simulink model "Driver"  (R2026b)
settings: Solver=VariableStepAuto
undefined symbols (not defined in the file): Driver, Maneuver, Scene, Vehicle, Visual, X, xy_data_car_side, Y, Z
libraries: sm_lib x18, simulink x13, nesl_utility x5, drivingvehiclecontroller x1, autolibshared x1, $bdroot x1
(part 2 of 2)

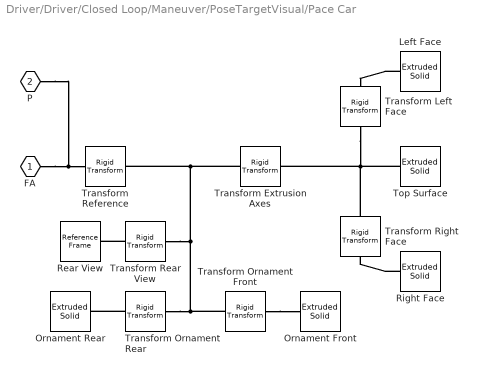
== system Driver/Driver/Closed Loop/Maneuver/PoseTargetVisual/Pace Car ==
  Left Face : sm_lib/Body Elements/Extruded Solid  ExtrusionType=General  PolygonNumSides=3  PolygonOuterRadius=1  PolygonOuterRadiusUnits=m  ExportEntireGeometry=off  ExtrusionCrossSection=xy_data_car_side  ExtrusionCrossSectionUnits=m  ExportConvexHullGeometry=off  ExtrusionLength=thk_side  ExtrusionLengthUnits=m  InertiaType=PointMass  BasedOnType=Density  Density=1000  DensityUnits=kg/m^3  Mass=0  MassUnits=kg  CenterOfMass=[0 0 0]  CenterOfMassUnits=m  MomentsOfInertia=[1 1 1]  MomentsOfInertiaUnits=kg*m^2  ProductsOfInertia=[0 0 0]  ProductsOfInertiaUnits=kg*m^2  GraphicType=FromGeometry  MarkerShape=Sphere  MarkerSize=10  GraphicVisPropType=SimpleVisualProperties  GraphicDiffuseColor=clr_body_geo_left  GraphicOpacity=opc_body_geo_left  GraphicSpecularColor=[0.5 0.5 0.5 1.0]  GraphicAmbientColor=[0.15 0.15 0.15 1.0]  GraphicEmissiveColor=[0.0 0.0 0.0 1.0]  GraphicShininess=75  DoExposeReferenceFrame=on  SerializedFrames=<Frames/>
  Ornament Front : sm_lib/Body Elements/Extruded Solid  ExtrusionType=General  PolygonNumSides=3  PolygonOuterRadius=1  PolygonOuterRadiusUnits=m  ExportEntireGeometry=off  ExtrusionCrossSection=extr_data_emblem_f  ExtrusionCrossSectionUnits=m  ExportConvexHullGeometry=off  ExtrusionLength=0.01  ExtrusionLengthUnits=m  InertiaType=CalculateFromGeometry  BasedOnType=Density  Density=1000  DensityUnits=kg/m^3  Mass=1  MassUnits=kg  CenterOfMass=[0 0 0]  CenterOfMassUnits=m  MomentsOfInertia=[1 1 1]  MomentsOfInertiaUnits=kg*m^2  ProductsOfInertia=[0 0 0]  ProductsOfInertiaUnits=kg*m^2  GraphicType=FromGeometry  MarkerShape=Sphere  MarkerSize=10  GraphicVisPropType=SimpleVisualProperties  GraphicDiffuseColor=clr_emblem_f  GraphicOpacity=opc_emblem_f  GraphicSpecularColor=[0.5 0.5 0.5 1.0]  GraphicAmbientColor=[0.15 0.15 0.15 1.0]  GraphicEmissiveColor=[0.0 0.0 0.0 1.0]  GraphicShininess=75  DoExposeReferenceFrame=on  SerializedFrames=<Frames/>
  Ornament Rear : sm_lib/Body Elements/Extruded Solid  ExtrusionType=General  PolygonNumSides=3  PolygonOuterRadius=1  PolygonOuterRadiusUnits=m  ExportEntireGeometry=off  ExtrusionCrossSection=extr_data_emblem_r  ExtrusionCrossSectionUnits=m  ExportConvexHullGeometry=off  ExtrusionLength=0.01  ExtrusionLengthUnits=m  InertiaType=CalculateFromGeometry  BasedOnType=Density  Density=1000  DensityUnits=kg/m^3  Mass=1  MassUnits=kg  CenterOfMass=[0 0 0]  CenterOfMassUnits=m  MomentsOfInertia=[1 1 1]  MomentsOfInertiaUnits=kg*m^2  ProductsOfInertia=[0 0 0]  ProductsOfInertiaUnits=kg*m^2  GraphicType=FromGeometry  MarkerShape=Sphere  MarkerSize=10  GraphicVisPropType=SimpleVisualProperties  GraphicDiffuseColor=clr_emblem_r  GraphicOpacity=opc_emblem_r  GraphicSpecularColor=[0.5 0.5 0.5 1.0]  GraphicAmbientColor=[0.15 0.15 0.15 1.0]  GraphicEmissiveColor=[0.0 0.0 0.0 1.0]  GraphicShininess=75  DoExposeReferenceFrame=on  SerializedFrames=<Frames/>
  Rear View : sm_lib/Frames and Transforms/Reference Frame
  Right Face : sm_lib/Body Elements/Extruded Solid  ExtrusionType=General  PolygonNumSides=3  PolygonOuterRadius=1  PolygonOuterRadiusUnits=m  ExportEntireGeometry=off  ExtrusionCrossSection=xy_data_car_side  ExtrusionCrossSectionUnits=m  ExportConvexHullGeometry=off  ExtrusionLength=thk_side  ExtrusionLengthUnits=m  InertiaType=PointMass  BasedOnType=Density  Density=1000  DensityUnits=kg/m^3  Mass=0  MassUnits=kg  CenterOfMass=[0 0 0]  CenterOfMassUnits=m  MomentsOfInertia=[1 1 1]  MomentsOfInertiaUnits=kg*m^2  ProductsOfInertia=[0 0 0]  ProductsOfInertiaUnits=kg*m^2  GraphicType=FromGeometry  MarkerShape=Sphere  MarkerSize=10  GraphicVisPropType=SimpleVisualProperties  GraphicDiffuseColor=clr_body_geo_right  GraphicOpacity=opc_body_geo_right  GraphicSpecularColor=[0.5 0.5 0.5 1.0]  GraphicAmbientColor=[0.15 0.15 0.15 1.0]  GraphicEmissiveColor=[0.0 0.0 0.0 1.0]  GraphicShininess=75  DoExposeReferenceFrame=on  SerializedFrames=<Frames/>
  Top Surface : sm_lib/Body Elements/Extruded Solid  ExtrusionType=General  PolygonNumSides=3  PolygonOuterRadius=1  PolygonOuterRadiusUnits=m  ExportEntireGeometry=off  ExtrusionCrossSection=xy_data_car_top  ExtrusionCrossSectionUnits=m  ExportConvexHullGeometry=off  ExtrusionLength=car_track  ExtrusionLengthUnits=m  InertiaType=PointMass  BasedOnType=Density  Density=0  DensityUnits=kg/m^3  Mass=0  MassUnits=kg  CenterOfMass=[0 0 0]  CenterOfMassUnits=m  MomentsOfInertia=[1 1 1]  MomentsOfInertiaUnits=kg*m^2  ProductsOfInertia=[0 0 0]  ProductsOfInertiaUnits=kg*m^2  GraphicType=FromGeometry  MarkerShape=Sphere  MarkerSize=10  GraphicVisPropType=SimpleVisualProperties  GraphicDiffuseColor=clr_body_geo_top  GraphicOpacity=opc_body_geo_top  GraphicSpecularColor=[0.5 0.5 0.5 1.0]  GraphicAmbientColor=[0.15 0.15 0.15 1.0]  GraphicEmissiveColor=[0.0 0.0 0.0 1.0]  GraphicShininess=75  DoExposeReferenceFrame=on  SerializedFrames=<Frames/>
  Transform Extrusion Axes : sm_lib/Frames and Transforms/Rigid Transform  RotationMethod=StandardAxis  FollAlignAxisA=+X  BaseAlignAxisA=+Y  FollAlignAxisB=+Y  BaseAlignAxisB=+Z  RotationStandardAxis=+X  RotationAngle=90  RotationAngleUnits=deg  RotationArbitraryAxis=[0 0 1]  RotationSequenceAxes=FollowerAxes  RotationSequence=XYX  RotationSequenceAngles=[0 0 0]  RotationSequenceAnglesUnits=deg  RotationMatrix=[1 0 0; 0 1 0; 0 0 1]  Quaternion=[1 0 0 0]  TranslationMethod=None  TranslationCartesianOffset=[0 0 0]  TranslationCartesianOffsetUnits=m  TranslationStandardAxis=+Z  TranslationStandardOffset=0  TranslationStandardOffsetUnits=m  TranslationROffset=0  TranslationROffsetUnits=m  TranslationThetaOffset=0  TranslationThetaOffsetUnits=deg  TranslationZOffset=0  TranslationZOffsetUnits=m
  Transform Ornament Front : sm_lib/Frames and Transforms/Rigid Transform  RotationMethod=RotationSequence  FollAlignAxisA=+X  BaseAlignAxisA=+Y  FollAlignAxisB=+Y  BaseAlignAxisB=+Z  RotationStandardAxis=+Z  RotationAngle=90  RotationAngleUnits=deg  RotationArbitraryAxis=[0 0 1]  RotationSequenceAxes=FollowerAxes  RotationSequence=ZXY  RotationSequenceAngles=[90 90 0]  RotationSequenceAnglesUnits=deg  RotationMatrix=[1 0 0; 0 1 0; 0 0 1]  Quaternion=[1 0 0 0]  TranslationMethod=Cartesian  TranslationCartesianOffset=[max(xy_data_car_side(:,1)) 0 min(xy_data_car_side(:,2))+0.15]  TranslationCartesianOffsetUnits=m  TranslationStandardAxis=+Z  TranslationStandardOffset=1  TranslationStandardOffsetUnits=m  TranslationROffset=0  TranslationROffsetUnits=m  TranslationThetaOffset=0  TranslationThetaOffsetUnits=deg  TranslationZOffset=0  TranslationZOffsetUnits=m
  Transform Ornament Rear : sm_lib/Frames and Transforms/Rigid Transform  RotationMethod=RotationSequence  FollAlignAxisA=+X  BaseAlignAxisA=+Y  FollAlignAxisB=+Y  BaseAlignAxisB=+Z  RotationStandardAxis=+Z  RotationAngle=90  RotationAngleUnits=deg  RotationArbitraryAxis=[0 0 1]  RotationSequenceAxes=FollowerAxes  RotationSequence=ZXY  RotationSequenceAngles=[90 90 180]  RotationSequenceAnglesUnits=deg  RotationMatrix=[1 0 0; 0 1 0; 0 0 1]  Quaternion=[1 0 0 0]  TranslationMethod=Cartesian  TranslationCartesianOffset=[min(xy_data_car_side(:,1))+0.1 0 min(xy_data_car_side(:,2))+0.15]  TranslationCartesianOffsetUnits=m  TranslationStandardAxis=+Z  TranslationStandardOffset=1  TranslationStandardOffsetUnits=m  TranslationROffset=0  TranslationROffsetUnits=m  TranslationThetaOffset=0  TranslationThetaOffsetUnits=deg  TranslationZOffset=0  TranslationZOffsetUnits=m
  Transform Rear View : sm_lib/Frames and Transforms/Rigid Transform  RotationMethod=None  FollAlignAxisA=+X  BaseAlignAxisA=+Y  FollAlignAxisB=+Y  BaseAlignAxisB=+Z  RotationStandardAxis=+Z  RotationAngle=0.0  RotationAngleUnits=deg  RotationArbitraryAxis=[0 0 1]  RotationSequenceAxes=FollowerAxes  RotationSequence=XYX  RotationSequenceAngles=[0 0 0]  RotationSequenceAnglesUnits=deg  RotationMatrix=[1 0 0; 0 1 0; 0 0 1]  Quaternion=[1 0 0 0]  TranslationMethod=Cartesian  TranslationCartesianOffset=[min(xy_data_car_side(:,1))-4 0 min(xy_data_car_side(:,2))+1]  TranslationCartesianOffsetUnits=m  TranslationStandardAxis=+Z  TranslationStandardOffset=0  TranslationStandardOffsetUnits=m  TranslationROffset=0  TranslationROffsetUnits=m  TranslationThetaOffset=0  TranslationThetaOffsetUnits=deg  TranslationZOffset=0  TranslationZOffsetUnits=m
  Transform Reference : sm_lib/Frames and Transforms/Rigid Transform  RotationMethod=None  FollAlignAxisA=+X  BaseAlignAxisA=+Y  FollAlignAxisB=+Y  BaseAlignAxisB=+Z  RotationStandardAxis=+Z  RotationAngle=0.0  RotationAngleUnits=deg  RotationArbitraryAxis=[0 0 1]  RotationSequenceAxes=FollowerAxes  RotationSequence=XYX  RotationSequenceAngles=[0 0 0]  RotationSequenceAnglesUnits=deg  RotationMatrix=[1 0 0; 0 1 0; 0 0 1]  Quaternion=[1 0 0 0]  TranslationMethod=Cartesian  TranslationCartesianOffset=offset_ref  TranslationCartesianOffsetUnits=m  TranslationStandardAxis=+Z  TranslationStandardOffset=0  TranslationStandardOffsetUnits=m  TranslationROffset=0  TranslationROffsetUnits=m  TranslationThetaOffset=0  TranslationThetaOffsetUnits=deg  TranslationZOffset=0  TranslationZOffsetUnits=m
  Transform Left Face : sm_lib/Frames and Transforms/Rigid Transform  RotationMethod=None  FollAlignAxisA=+X  BaseAlignAxisA=+Y  FollAlignAxisB=+Y  BaseAlignAxisB=+Z  RotationStandardAxis=+Z  RotationAngle=0.0  RotationAngleUnits=deg  RotationArbitraryAxis=[0 0 1]  RotationSequenceAxes=FollowerAxes  RotationSequence=XYX  RotationSequenceAngles=[0 0 0]  RotationSequenceAnglesUnits=deg  RotationMatrix=[1 0 0; 0 1 0; 0 0 1]  Quaternion=[1 0 0 0]  TranslationMethod=StandardAxis  TranslationCartesianOffset=[0 0 0]  TranslationCartesianOffsetUnits=m  TranslationStandardAxis=-Z  TranslationStandardOffset=car_track/2-thk_side/2  TranslationStandardOffsetUnits=m  TranslationROffset=0  TranslationROffsetUnits=m  TranslationThetaOffset=0  TranslationThetaOffsetUnits=deg  TranslationZOffset=0  TranslationZOffsetUnits=m
  Transform Right Face : sm_lib/Frames and Transforms/Rigid Transform  RotationMethod=None  FollAlignAxisA=+X  BaseAlignAxisA=+Y  FollAlignAxisB=+Y  BaseAlignAxisB=+Z  RotationStandardAxis=+Z  RotationAngle=0.0  RotationAngleUnits=deg  RotationArbitraryAxis=[0 0 1]  RotationSequenceAxes=FollowerAxes  RotationSequence=XYX  RotationSequenceAngles=[0 0 0]  RotationSequenceAnglesUnits=deg  RotationMatrix=[1 0 0; 0 1 0; 0 0 1]  Quaternion=[1 0 0 0]  TranslationMethod=StandardAxis  TranslationCartesianOffset=[0 0 0]  TranslationCartesianOffsetUnits=m  TranslationStandardAxis=+Z  TranslationStandardOffset=car_track/2-thk_side/2  TranslationStandardOffsetUnits=m  TranslationROffset=0  TranslationROffsetUnits=m  TranslationThetaOffset=0  TranslationThetaOffsetUnits=deg  TranslationZOffset=0  TranslationZOffsetUnits=m
  FA : PMIOPort  Side=Right
  P : PMIOPort  Port=2  Side=Left
  connections:
  Transform Ornament Rear/RConn1 -- Ornament Rear/RConn1
  Transform Ornament Front/RConn1 -- Ornament Front/RConn1
  Right Face/RConn1 -- Transform Right Face/RConn1
  Transform Left Face/LConn1 -- Top Surface/RConn1 -- Transform Right Face/LConn1 -- Transform Extrusion Axes/RConn1
  Left Face/RConn1 -- Transform Left Face/RConn1
  Transform Extrusion Axes/LConn1 -- Transform Reference/RConn1 -- Transform Rear View/LConn1 -- Transform Ornament Rear/LConn1 -- Transform Ornament Front/LConn1
  Transform Rear View/RConn1 -- Rear View/RConn1
  FA/RConn1 -- P/RConn1 -- Transform Reference/LConn1

== system Driver/Driver/Closed Loop/Maneuver/PoseTargetVisual/Count Lap/Triggered Subsystem ==
  Up Down : Inport
  Trigger : TriggerPort  VariantControl=Variant  ZeroCross=off
  Memory : Memory  InheritSampleTime=on
  Sum : Sum  Inputs=|++
  Num Laps : Outport  VectorParamsAs1DForOutWhenUnconnected=off
  wires:
  Memory/1 -> Sum/1
  Sum/1 -> Memory/1, Num Laps/1
  Up Down/1 -> Sum/2

== matlab function Driver/Closed Loop/Maneuver/MATLAB Function ==
  data: ad output; ref_z output; ref_x output; ref_y output; ref_ayaw output; vTarget output; cp output; p input; q input; posx input; posy input; posz input; xywin input; speed input; yaw input; dist input; pd input; maxld input; minSpd input; speedGain input; ld output; idx_ptMin output; simres output; idx_ptMin_prev input
function [ad,ref_z,ref_x,ref_y,ref_ayaw,vTarget,cp,ld, idx_ptMin, simres] = getPoseCurRef(p,q,posx,posy,posz,xywin,speed,yaw,dist,pd, maxld, minSpd, speedGain, idx_ptMin_prev)

% This function determines the target pose for the vehicle.  It
% interpolates within the provided trajectory to determine the target
% x-y position, yaw angle, and speed. The targets are defined with respect
% to distance along the target trajectory.  The first portion of the
% function determines the distance along the trajectory that the vehicle
% has traveled (ad).  Once that is found, the function interpolates to find
% the target pose at the preview distance (ad+pd).

npts = length(posx);

% Look for nearest point in a window near last evaluation
% Obtain window
if (idx_ptMin_prev == -1)
    % For first evaluation, use entire list of points
    ptlist = 1:npts;
elseif((idx_ptMin_prev-xywin)<1)
    % Window overlaps at lower end: take points from upper end
    win2 = (npts+idx_ptMin_prev-xywin):1:npts;
    win1 = 1:(idx_ptMin_prev+xywin);
    ptlist = [win1 win2];
elseif((idx_ptMin_prev+xywin)>npts)
    % Window overlaps at upper end: take points from lower end
    win2 = (idx_ptMin_prev-xywin):1:npts;
    win1 = 1:(idx_ptMin_prev+xywin-npts);
    ptlist = [win1 win2];
else
    % No overlap: use window
    ptlist = (idx_ptMin_prev-xywin):1:(idx_ptMin_prev+xywin);
end

% Find closest supplied trajectory point to current car position
distances = hypot(p(1) - posx,p(2) - posy);
distances_srch = distances(ptlist);
[~, idx_ptlist] = min(distances_srch);
idx_ptMin = ptlist(idx_ptlist);

%% Identify two trajectory points ahead of and behind closest supplied point
% A, B, C (closest), D, E
idx_ptC = idx_ptMin;
idx_ptA = idx_ptMin-2;
idx_ptB = idx_ptMin-1;
idx_ptD = idx_ptMin+1;
idx_ptE = idx_ptMin+2;

% If we are at end of trajectory, wrap point index
if (idx_ptA<=0),   idx_ptA = idx_ptA+npts; end
if (idx_ptB<=0),   idx_ptB = idx_ptB+npts; end
if (idx_ptD>npts), idx_ptD = idx_ptD-npts; end
if (idx_ptE>npts), idx_ptE = idx_ptE-npts; end

% Extract trajectory point x-y locations
ptA = [posx(idx_ptA); posy(idx_ptA)];
ptB = [posx(idx_ptB); posy(idx_ptB)];
ptC = [posx(idx_ptC); posy(idx_ptC)];
ptD = [posx(idx_ptD); posy(idx_ptD)];
ptE = [posx(idx_ptE); posy(idx_ptE)];

%% Find line separating trajectory segments BC, CD
% Find angle of line connecting BD
qBD = atan2(ptD(2)-ptB(2),ptD(1)-ptB(1));

% Angle of line separating BC, CD is normal to that line
qC  = qBD+pi/2;

%% Determine if we are nearest to trajectory segment BC or BD
% Check if vehicle location and point B on same side of line
% separating segments BC and BD
segBC = arePointsOnSameSide(ptC(1), ptC(2), tan(qC), p(1), p(2), ptB(1), ptB(2));

%% Find vehicle line segment 
% Segment is parallel to closest trajectory segment on which vehicle lies
if(segBC)
   % Use segment BC
   % Line dividing segments AB and BC is normal to line AC 
   qR = atan2(ptC(2)-ptA(2),ptC(1)-ptA(1))+pi/2;
   % Line dividing segments BC and CD has already been found 
   qF = qC;

   ptR = ptB;  % Rear point of segment is point B
   ptF = ptC;  % Front point of segment is point C

   % Angle of vehicle line segment is same as angle of segment BC
   qV = atan2(ptC(2)-ptB(2),ptC(1)-ptB(1));
    % Distance along trajectory to rear of segment
   distR    = dist(idx_ptB);
else
   % Use segment CD
   % Line dividing segments BC and CD has already been found 
   qR = qC;
   % Line dividing segments CD and DE is normal to line CE 
   qF = atan2(ptE(2)-ptC(2),ptE(1)-ptC(1))+pi/2;

   ptR = ptC;    % Rear point of segment is point B
   ptF = ptD;    % Front point of segment is point C

   % Angle of vehicle line segment is same as angle of segment CD
   qV = atan2(ptD(2)-ptC(2),ptD(1)-ptC(1));
    % Distance along trajectory to rear of segment
   distR = dist(idx_ptC);
end

% Length of trajectory segment
distSeg  = sqrt((ptF(1)-ptR(1))^2+(ptF(2)-ptR(2))^2);

% Find endpoints of vehicle line segment
[xR, yR] = findIntersection(p(1), p(2), tan(qV), ptR(1), ptR(2), tan(qR));
[xF, yF] = findIntersection(p(1), p(2), tan(qV), ptF(1), ptF(2), tan(qF));

% Length of vehicle line segment
distFR = sqrt((xR-xF)^2+(yR-yF)^2);
% Distance of vehicle location from rear of vehicle line segment
distvR = sqrt((xR-p(1))^2+(yR-p(2))^2);

% Percentage of distance from vehicle to rear of vehicle line segment 
% Do not permit percentage to go above 100%
% Occurs when vehicle is far from line on inside of curve
segPcnt = min(distvR/distFR,1);

% Distance along trajectory = 
%   Distance to rear of trajectory segment + 
%   length of closest trajectory segment * 
%   percent of vehicle line segment already completed
ad = distR+segPcnt*distSeg;

% Find angle between vehicle location, forward point, and track trajectory
vec_F2v  = ptF - [p(1); p(2)];
vec_F2R  = ptF - ptR;

% Use cosine formula to obtain angle
cos_ang_new = dot(vec_F2v,vec_F2R)/(norm(vec_F2v)*norm(vec_F2R));

% Bound cosine of angle between eps and 1
cos_ang_new = max(cos_ang_new,eps);
cos_ang_new = min(cos_ang_new,1-eps);

% Use angle to obtain lateral distance of vehicle from trajectory
ld = norm(vec_F2v)*sin(acos(cos_ang_new));

% Pose targets for Stanley controller (distance cumulatively sums)
dist4interp = [-dist(end)+dist(1:end-1); dist; dist(end)+dist(2:end)];
posx4interp = [           posx(1:end-1); posx;           posx(2:end)];
posy4interp = [           posy(1:end-1); posy;           posy(2:end)];
posz4interp = [           posz(1:end-1); posz;           posz(2:end)];
speed4interp= [          speed(1:end-1);speed;          speed(2:end)];
% Wrap the interpolation vector for yaw.  
% Necessary to avoid obtaining values between yaw(end) and yaw(1)
yaw4interp  = [-(yaw(end)-yaw(1)) + yaw(1:end-1);  yaw;  (yaw(end)-yaw(1))+ yaw(2:end)];

% Current point
cp = [p(1);p(2);q(3)*180/pi]';

% Reference point obtained from supplied trajectory
% Interpolate using Actual distance (ad) + preview distance (pd)
ref_x    = interp1(dist4interp,posx4interp,ad+pd,'pchip');
ref_y    = interp1(dist4interp,posy4interp,ad+pd,'pchip');
ref_ayaw = interp1(dist4interp,yaw4interp, ad+pd,'pchip');

% For visualization only
ref_z    = interp1(dist4interp,posz4interp,ad+pd);

% Reference velocity obtained from supplied trajectory
% Interpolate using actual distance
vx_cp = interp1(dist4interp,speed4interp,ad);

% Protect for NaNs
ref_x(isnan(ref_x)) = 0;
ref_y(isnan(ref_y)) = 0;
ref_ayaw(isnan(ref_ayaw)) = 0;
ref_z(isnan(ref_z)) = 0;

% Scale speed target
% Reduce speed target if car is far from the target trajectory
if ld < maxld
    vTarget = vx_cp * speedGain;
else
    vTarget = minSpd;
end

% Outputs for debugging calculation
simres = [idx_ptA idx_ptB idx_ptC idx_ptD idx_ptE qC segBC segPcnt xR yR  xF yF p(1) p(2) ad distR distSeg];

end

function [x_intersect, y_intersect] = findIntersection(x1, y1, m1, x2, y2, m2)
    % Check if the slopes are equal (parallel lines)
    if m1 == m2
        error('Invalid trajectory points. The lines are parallel and do not intersect.');
    end
    
    % Calculate the intersection point
    x_intersect = (y2 - y1 + m1*x1 - m2*x2) / (m1 - m2);
    y_intersect = m1 * (x_intersect - x1) + y1;
end

function same_side = arePointsOnSameSide(x0, y0, m, x1, y1, x2, y2)
    % Calculate the line coefficients
    a = -m; % Coefficient of x
    b = 1;  % Coefficient of y
    c = m*x0 - y0; % Constant term
    
    % Calculate the line equation value for both points
    value1 = a*x1 + b*y1 + c;
    value2 = a*x2 + b*y2 + c;
    
    % Check if both values have the same sign
    same_side = (value1 * value2) > 0;
end
